simulink model "AWU_back_calculation"  (R2023a)
settings: Solver=VariableStepAuto  StartTime=0.0  StopTime=60  RelTol=1e-3
values from neighbouring files (symbols this model uses):
  lower_limit = -0.2    [AWU_system_data.sldd]
  upper_limit = 0.2    [AWU_system_data.sldd]
undefined symbols (not defined in the file or in its folder): DiscIntNeverNeededParam
libraries: simulink x1, SignalEditorBlockLib x1
settings Model: DataDictionary=AWU_system_data.sldd  Creator=tshintai  LastModifiedBy=tshintai
settings SolverCC: AlgebraicLoopSolver=TrustRegion
settings OptimizationCC: ReuseModelBlockBuffer=off
settings DebuggingCC: UnconnectedInputMsg=warning  UnconnectedOutputMsg=warning  UnconnectedLineMsg=warning
settings ModelReferenceCC: EnableRefExpFcnMdlSchedulingChecks=on
settings RTWCC: DLArmComputeVersion=19.05

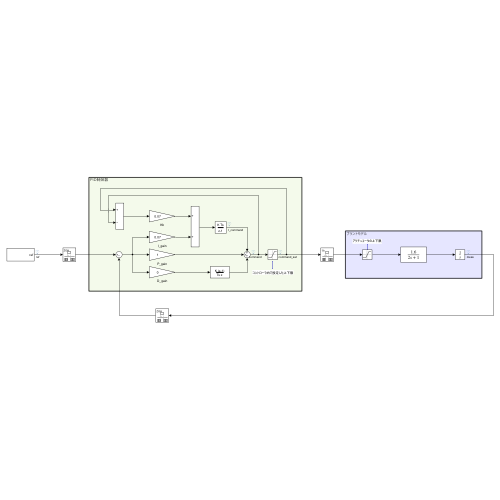
[thumbnail: Simulink's stored preview of the top-level diagram]
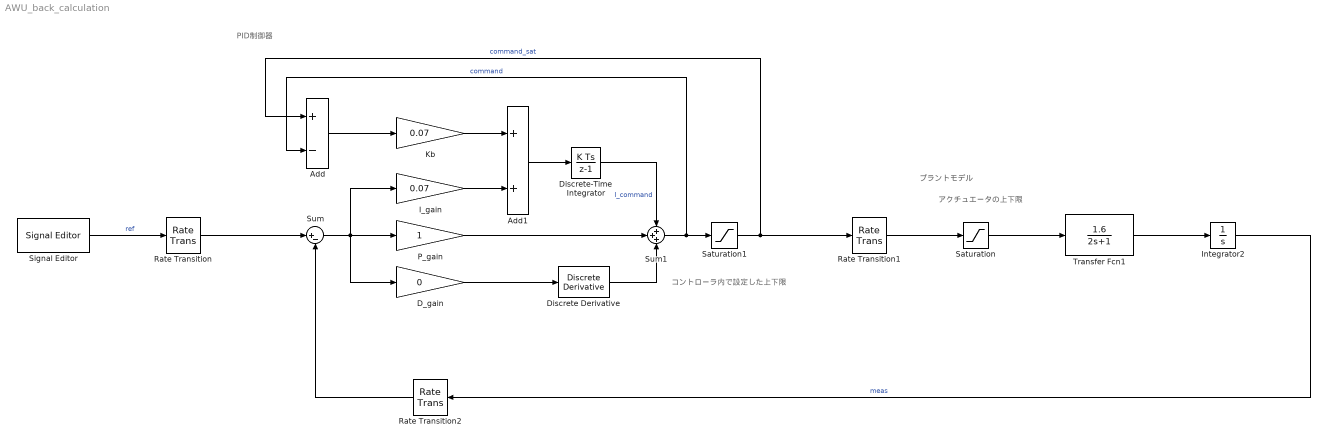
== system AWU_back_calculation ==
  note: PID制御器
  note: アクチュエータの上下限
  note: プラントモデル
  note: コントローラ内で設定した上下限
  Add : Sum  Inputs=+-
  Add1 : Sum
  D_gain : Gain  Gain=0
  Discrete Derivative : simulink/Discrete/Discrete Derivative  gainval=1.0  ICPrevScaledInput=0.0  OutMin=[]  OutMax=[]  OutDataType=fixdt(1, 16)  OutScaling=2^-10  DoSatur=off
  Discrete-Time Integrator : DiscreteIntegrator  SampleTime=-1  ICPrevOutput=DiscIntNeverNeededParam  ICPrevScaledInput=DiscIntNeverNeededParam
  I_gain : Gain  Gain=0.07
  Integrator2 : Integrator
  Kb : Gain  Gain=0.07
  P_gain : Gain
  Rate Transition : RateTransition  OutPortSampleTime=TimeStep
  Rate Transition1 : RateTransition
  Rate Transition2 : RateTransition  OutPortSampleTime=TimeStep
  Saturation : Saturate  UpperLimit=0.2  LowerLimit=-0.2
  Saturation1 : Saturate  UpperLimit=upper_limit  LowerLimit=lower_limit
  Signal Editor : SignalEditorBlockLib/Signal Editor  FileName=AWU_ref_signal.mat  ActiveScenario=Scenario  ActiveSignal=ref  IsBus=off  OutputBusObjectStr=Bus: BusObject  SampleTime=0  ZeroCross=off  OutputAfterFinalValue=Holding final value  Unit=inherit  PreserveSignalName=on  ApplySigPropsToAllScenarios=on
  Sum : Sum  Inputs=|+-
  Sum1 : Sum  Inputs=+++
  Transfer Fcn1 : TransferFcn  Numerator=[1.6]  Denominator=[2 1]
  wires:
  Transfer Fcn1/1 -> Integrator2/1
  Saturation/1 -> Transfer Fcn1/1
  Integrator2/1 -> Rate Transition2/1  "meas"
  Sum/1 -> D_gain/1, I_gain/1, P_gain/1
  D_gain/1 -> Discrete Derivative/1
  P_gain/1 -> Sum1/2
  Discrete Derivative/1 -> Sum1/3
  Saturation1/1 -> Add/1, Rate Transition1/1  "command_sat"
  Signal Editor/1 -> Rate Transition/1  "ref"
  Rate Transition/1 -> Sum/1
  Rate Transition1/1 -> Saturation/1
  Rate Transition2/1 -> Sum/2
  Sum1/1 -> Add/2, Saturation1/1  "command"
  I_gain/1 -> Add1/2
  Discrete-Time Integrator/1 -> Sum1/1  "I_command"
  Add/1 -> Kb/1
  Kb/1 -> Add1/1
  Add1/1 -> Discrete-Time Integrator/1
